simulink model "SolarMicrogrid"  (R2023a)
settings: Solver=FixedStepDiscrete  StartTime=0.0  StopTime=86400  FixedStep=1  RelTol=1e-3
PostLoadFcn:
  | run(fullfile(fileparts(get_param('SolarMicrogrid','FileName')),'microgrid_params.m'));
InitFcn:
  | run(fullfile(fileparts(get_param('SolarMicrogrid','FileName')),'microgrid_params.m'));
undefined symbols (not defined in the file or in its folder): DiscIntNeverNeededParam, P
settings Model: Creator=samir mallick  LastModifiedBy=samir mallick

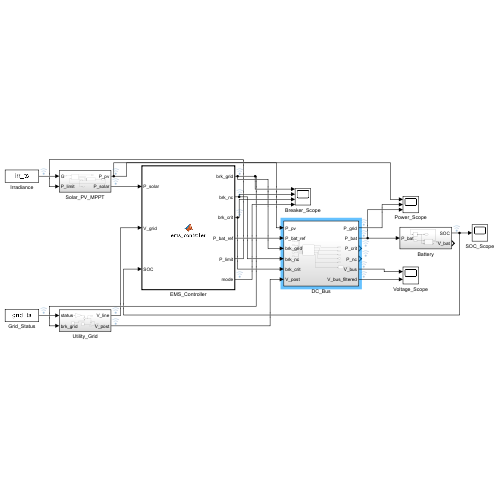
[thumbnail: Simulink's stored preview of the top-level diagram]
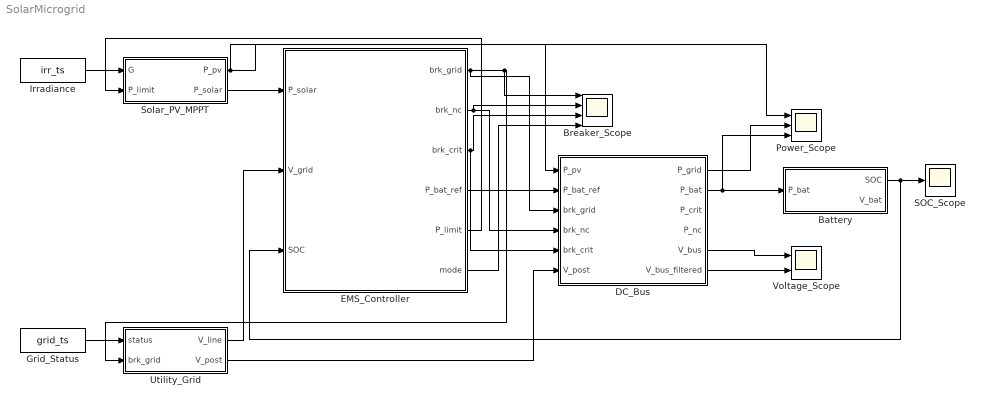
== system SolarMicrogrid ==
  Battery : Subsystem
  Breaker_Scope : Scope  NumInputPorts=4
  DC_Bus : Subsystem
  EMS_Controller : MATLAB Function  TreatAsAtomicUnit=on
  Grid_Status : FromWorkspace  VariableName=grid_ts  Interpolate=off  OutputAfterFinalValue=Holding final value
  Irradiance : FromWorkspace  VariableName=irr_ts
  Power_Scope : Scope  NumInputPorts=3
  SOC_Scope : Scope
  Solar_PV_MPPT : Subsystem
  Utility_Grid : Subsystem
  Voltage_Scope : Scope  NumInputPorts=2
  wires:
  EMS_Controller/1(brk_grid) -> Utility_Grid/2(brk_grid), Breaker_Scope/1, DC_Bus/3(brk_grid)
  Irradiance/1 -> Solar_PV_MPPT/1(G)
  DC_Bus/6(V_bus_filtered) -> Voltage_Scope/2
  Utility_Grid/2(V_post) -> DC_Bus/6(V_post)
  DC_Bus/2(P_bat) -> Battery/1(P_bat), Power_Scope/3
  Utility_Grid/1(V_line) -> EMS_Controller/2(V_grid)
  DC_Bus/5(V_bus) -> Voltage_Scope/1
  Grid_Status/1 -> Utility_Grid/1(status)
  Solar_PV_MPPT/1(P_pv) -> DC_Bus/1(P_pv), Power_Scope/1
  Battery/1(SOC) -> SOC_Scope/1, EMS_Controller/3(SOC)
  Solar_PV_MPPT/2(P_solar) -> EMS_Controller/1(P_solar)
  EMS_Controller/2(brk_nc) -> DC_Bus/4(brk_nc), Breaker_Scope/2
  EMS_Controller/3(brk_crit) -> DC_Bus/5(brk_crit), Breaker_Scope/3
  EMS_Controller/4(P_bat_ref) -> DC_Bus/2(P_bat_ref)
  EMS_Controller/5(P_limit) -> Solar_PV_MPPT/2(P_limit)
  EMS_Controller/6(mode) -> Breaker_Scope/4
  DC_Bus/1(P_grid) -> Power_Scope/2

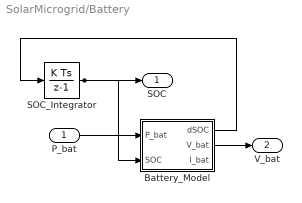
== system SolarMicrogrid/Battery ==
  P_bat : Inport
  Battery_Model : MATLAB Function  TreatAsAtomicUnit=on
  SOC_Integrator : DiscreteIntegrator  InitialCondition=P.SOC0  SampleTime=-1  LimitOutput=on  UpperSaturationLimit=1  LowerSaturationLimit=0  ICPrevOutput=DiscIntNeverNeededParam  ICPrevScaledInput=DiscIntNeverNeededParam
  SOC : Outport
  V_bat : Outport  Port=2
  wires:
  SOC_Integrator/1 -> Battery_Model/2(SOC), SOC/1
  P_bat/1 -> Battery_Model/1(P_bat)
  Battery_Model/1(dSOC) -> SOC_Integrator/1
  Battery_Model/2(V_bat) -> V_bat/1

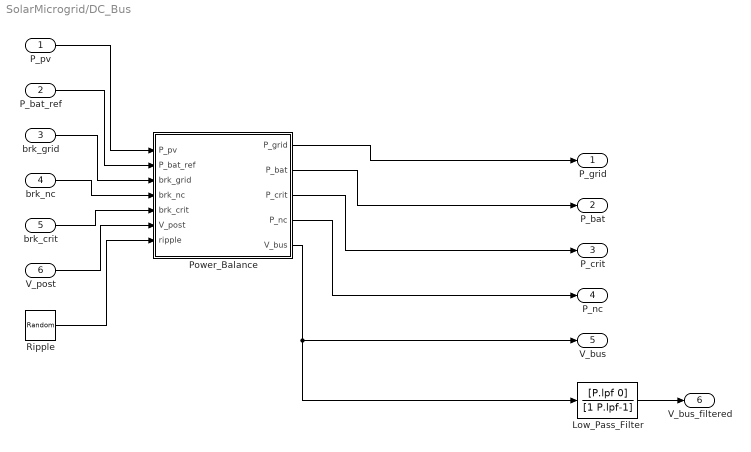
== system SolarMicrogrid/DC_Bus ==
  P_pv : Inport
  P_bat_ref : Inport  Port=2
  brk_grid : Inport  Port=3
  brk_nc : Inport  Port=4
  brk_crit : Inport  Port=5
  V_post : Inport  Port=6
  Low_Pass_Filter : DiscreteTransferFcn  Numerator=[P.lpf 0]  Denominator=[1 P.lpf-1]  InitialStates=12/P.lpf
  Power_Balance : MATLAB Function  TreatAsAtomicUnit=on
  Ripple : RandomNumber  Variance=P.noise^2  SampleTime=1
  P_grid : Outport
  P_bat : Outport  Port=2
  P_crit : Outport  Port=3
  P_nc : Outport  Port=4
  V_bus : Outport  Port=5
  V_bus_filtered : Outport  Port=6
  wires:
  P_pv/1 -> Power_Balance/1(P_pv)
  P_bat_ref/1 -> Power_Balance/2(P_bat_ref)
  V_post/1 -> Power_Balance/6(V_post)
  brk_crit/1 -> Power_Balance/5(brk_crit)
  brk_nc/1 -> Power_Balance/4(brk_nc)
  brk_grid/1 -> Power_Balance/3(brk_grid)
  Ripple/1 -> Power_Balance/7(ripple)
  Power_Balance/1(P_grid) -> P_grid/1
  Power_Balance/3(P_crit) -> P_crit/1
  Power_Balance/2(P_bat) -> P_bat/1
  Power_Balance/4(P_nc) -> P_nc/1
  Power_Balance/5(V_bus) -> Low_Pass_Filter/1, V_bus/1
  Low_Pass_Filter/1 -> V_bus_filtered/1

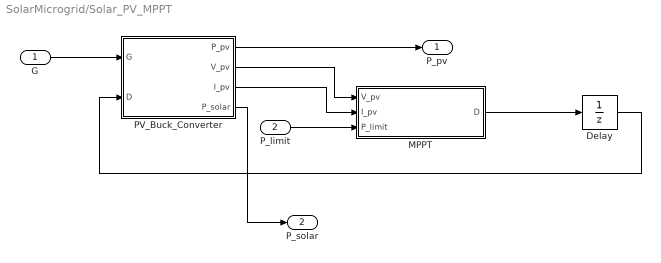
== system SolarMicrogrid/Solar_PV_MPPT ==
  G : Inport
  P_limit : Inport  Port=2
  Delay : UnitDelay  InitialCondition=P.D0  SampleTime=-1  HasFrameUpgradeWarning=on
  MPPT : MATLAB Function  TreatAsAtomicUnit=on
  PV_Buck_Converter : MATLAB Function  TreatAsAtomicUnit=on
  P_pv : Outport
  P_solar : Outport  Port=2
  wires:
  G/1 -> PV_Buck_Converter/1(G)
  PV_Buck_Converter/1(P_pv) -> P_pv/1
  PV_Buck_Converter/2(V_pv) -> MPPT/1(V_pv)
  PV_Buck_Converter/4(P_solar) -> P_solar/1
  PV_Buck_Converter/3(I_pv) -> MPPT/2(I_pv)
  P_limit/1 -> MPPT/3(P_limit)
  MPPT/1(D) -> Delay/1
  Delay/1 -> PV_Buck_Converter/2(D)

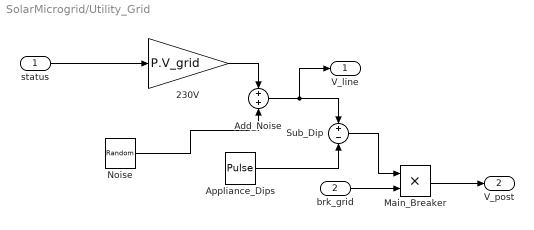
== system SolarMicrogrid/Utility_Grid ==
  status : Inport
  brk_grid : Inport  Port=2
  230V : Gain  Gain=P.V_grid
  Add_Noise : Sum
  Appliance_Dips : DiscretePulseGenerator  Amplitude=P.dip  Period=7200  PulseWidth=4  PhaseDelay=1800
  Main_Breaker : Product
  Noise : RandomNumber  Variance=4  SampleTime=1
  Sub_Dip : Sum  Inputs=+-
  V_line : Outport
  V_post : Outport  Port=2
  wires:
  Main_Breaker/1 -> V_post/1
  status/1 -> 230V/1
  brk_grid/1 -> Main_Breaker/2
  230V/1 -> Add_Noise/1
  Add_Noise/1 -> Sub_Dip/1, V_line/1
  Noise/1 -> Add_Noise/2
  Sub_Dip/1 -> Main_Breaker/1
  Appliance_Dips/1 -> Sub_Dip/2

== matlab function SolarMicrogrid/Solar_PV_MPPT/MPPT ==
  data: V_pv input; D output; I_pv input; P_limit input; P parameter
function D = mppt_po(V_pv, I_pv, P_limit, P)
% Perturb and Observe MPPT
% if the EMS gives a power limit (battery full) the duty is reduced so the
% panel gives less power

persistent D_old P_old step
if isempty(D_old)
    D_old = P.D0;
    P_old = 0;
    step = -P.dD;
end

P_now = P.eff*V_pv*I_pv;

if P_now < 1
    D = P.D0;                  % night time
elseif P_now > P_limit
    D = D_old - P.dD;          % too much power, move away from MPP
    step = P.dD;
elseif P_now > P_limit - 5
    D = D_old;                 % close enough to the limit, keep D
else
    if P_now < P_old
        step = -step;          % power went down so change direction
    end
    D = D_old + step;
end

D = min(max(D, P.D_min), P.D_max);

D_old = D;
P_old = P_now;
end

== matlab function SolarMicrogrid/Solar_PV_MPPT/PV_Buck_Converter ==
  data: G input; P_pv output; D input; V_pv output; I_pv output; P_solar output; P parameter
function [P_pv, V_pv, I_pv, P_solar] = pv_buck(G, D, P)
% Solar panel (single diode model) + buck converter
% for a buck converter Vout = D*Vin, so the panel voltage is Vpv = Vbus/D

G = max(G, 0);
Iph = P.Isc*G/1000;            % light generated current

D = min(max(D, P.D_min), P.D_max);
V_pv = P.V_bus/D;
I_pv = Iph - P.I0*(exp(V_pv/P.a) - 1);
if I_pv < 0
    I_pv = 0;                  % blocking diode
end

P_pv = P.eff*V_pv*I_pv;        % power going into the 12V bus

% available solar power estimated from irradiance (used by the EMS)
P_solar = P.P_rated*G/1000;
end

== matlab function SolarMicrogrid/Battery/Battery_Model ==
  data: P_bat input; dSOC output; SOC input; V_bat output; I_bat output; P parameter
function [dSOC, V_bat, I_bat] = battery_model(P_bat, SOC, P)
% simple battery model
% P_bat +ve = charging, -ve = discharging

Voc = P.Vb_min + (P.Vb_max - P.Vb_min)*SOC;   % open circuit voltage
I_bat = P_bat/Voc;
V_bat = Voc + I_bat*P.R_bat;

% coulomb counting
if I_bat > 0
    dSOC = P.eff_bat*I_bat/(3600*P.Ah);
else
    dSOC = I_bat/(P.eff_bat*3600*P.Ah);
end
end

== matlab function SolarMicrogrid/EMS_Controller ==
  data: P_solar input; brk_grid output; V_grid input; SOC input; brk_nc output; brk_crit output; P_bat_ref output; P_limit output; mode output; P parameter
function [brk_grid, brk_nc, brk_crit, P_bat_ref, P_limit, mode] = ems_controller(P_solar, V_grid, SOC, P)
% Energy Management System
% inputs : P_solar = solar power available (W), V_grid = grid voltage (V), SOC
% outputs: breaker signals (1 = closed), battery power reference
%          (+ve charge, -ve discharge), PV power limit for MPPT, mode
%
% mode 1 : grid ok, solar > load  -> solar feeds load, extra charges battery
% mode 2 : grid ok, solar < load  -> grid gives the rest + trickle charge
% mode 3 : blackout, solar > load -> solar feeds load, extra charges battery
% mode 4 : blackout, solar < load -> switch off non critical, battery feeds critical
% mode 5 : blackout, SOC <= 20%   -> battery cut off to protect it

persistent Vf full
if isempty(Vf)
    Vf = P.V_grid;
    full = 0;
end

% filter the grid voltage so noise does not cause false trips
Vf = Vf + P.alpha*(V_grid - Vf);
grid_ok = Vf > P.V_trip;

P_load = P.P_crit + P.P_nc;

% battery full flag (with hysteresis so it does not keep switching at 95%)
if SOC >= P.SOC_max
    full = 1;
elseif SOC < P.SOC_max - 0.05
    full = 0;
end

if full == 1
    P_chg = 0;
else
    P_chg = P.P_chg_max;
end

brk_grid = 1;
brk_nc = 1;
brk_crit = 1;

if grid_ok
    if P_solar >= P_load
        mode = 1;
        P_bat_ref = min(P_solar - P_load, P_chg);
    else
        mode = 2;
        P_bat_ref = min(P.P_trickle, P_chg);
    end
    P_limit = P_load + P_bat_ref;

else
    brk_grid = 0;   % open main breaker (islanded)

    if P_solar >= P_load
        mode = 3;
        P_bat_ref = min(P_solar - P_load, P_chg);
        P_limit = P_load + P_bat_ref;

    elseif SOC > P.SOC_min
        mode = 4;
        brk_nc = 0;     % load shedding
        P_bat_ref = min(P_solar - P.P_crit, P_chg);   % negative = discharge
        P_limit = P.P_crit + max(P_bat_ref, 0);

    else
        mode = 5;
        brk_nc = 0;
        if P_solar < P.P_crit
            brk_crit = 0;   % not enough power even for critical load
        end
        P_bat_ref = 0;
        P_limit = brk_crit*P.P_crit;
    end
end
end

== matlab function SolarMicrogrid/DC_Bus/Power_Balance ==
  data: P_pv input; P_grid output; P_bat_ref input; brk_grid input; brk_nc input; brk_crit input; V_post input; ripple input; P_bat output; P_crit output; P_nc output; V_bus output; P parameter
function [P_grid, P_bat, P_crit, P_nc, V_bus] = dc_bus(P_pv, P_bat_ref, brk_grid, brk_nc, brk_crit, V_post, ripple, P)
% power balance at the 12V DC bus
% grid connected -> grid supplies whatever is missing
% islanded       -> battery supplies whatever is missing

P_crit = brk_crit*P.P_crit;
P_nc = brk_nc*P.P_nc;
P_load = P_crit + P_nc;

if brk_grid == 1 && V_post > 100
    P_grid = P_load + P_bat_ref - P_pv;
    P_grid = min(max(P_grid, 0), P.P_grid_max);
    P_bat = P_pv + P_grid - P_load;
else
    P_grid = 0;
    P_bat = P_pv - P_load;
end

% bus voltage with some converter ripple (0 if all loads are off)
if P_load > 0
    V_bus = P.V_bus + ripple;
else
    V_bus = 0;
end
end
